simulink model "projeto_bateria_carro_eletrico"  (R2025b)
settings: Solver=VariableStepAuto  StartTime=0.0  StopTime=3600  MaxStep=0.1  RelTol=1e-3
model workspace (MAT data in the model file):
  Fr = 225
  Fr1 = 225
  Fr2 = 450
  Fr3 = 700
  Ft = 1
  V = 100
  t = 4
  v = 38.8888888889
undefined symbols (not defined in the file): Chart, Freio_regenerativo
settings Model: Creator=lucas russo  LastModifiedBy=lucas russo

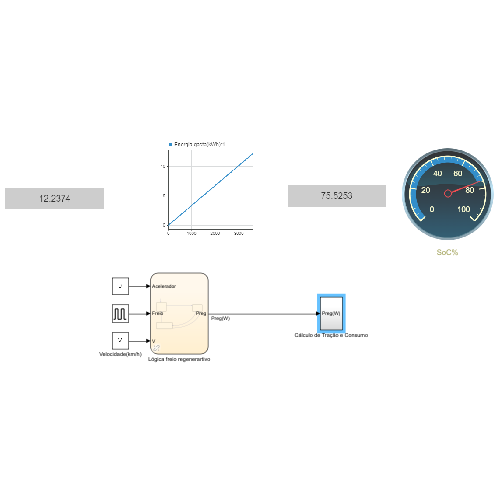
[thumbnail: Simulink's stored preview of the top-level diagram]
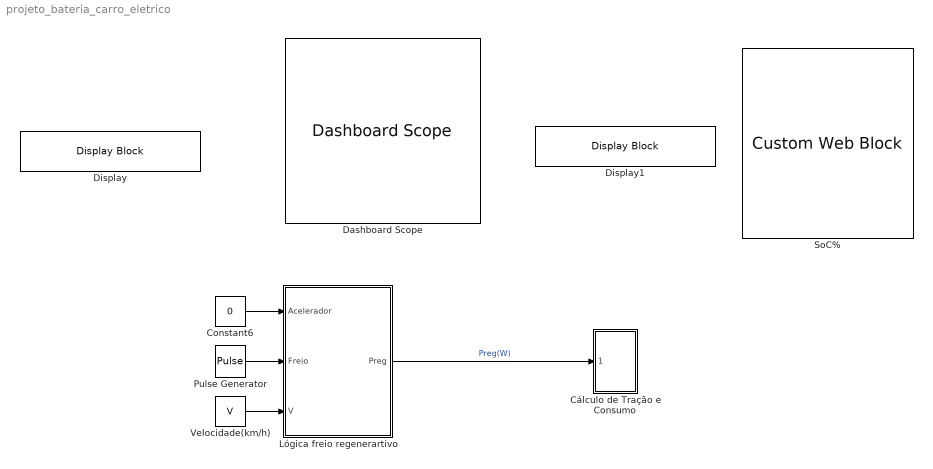
== system projeto_bateria_carro_eletrico ==
  Constant6 : Constant  Value=0
  Cálculo de Tração e Consumo : Subsystem
  Dashboard Scope : DashboardScope  Ymin=0  Ymax=50  FontColor=[0.0, 0.0, 0.0]
  Display : DisplayBlock  LabelPosition=Hide  Transparency=1  GridColor=[0.502, 0.502, 0.502]
  Display1 : DisplayBlock  LabelPosition=Hide  Transparency=1  GridColor=[0.502, 0.502, 0.502]
  Lógica freio regenerartivo : Stateflow chart  AncestorBlock=Freio_regenerativo/Chart
  Pulse Generator : DiscretePulseGenerator  PulseType=Time based  Period=360
  SoC% : CustomWebBlock  LabelPosition=Hide  ShowInitialText=on  Configuration="{\"components\":[{\"name\":\"CircularScaleComponent\",\"settings\":{\"bounds\":{\"max\":100,\"min\":0,\"tickInterval\":\"auto\"},\"direction\":\"cw\",\"flipLimits\":0,\"innerRadius\":0.75,\"internalTickHeightScaleFactor\":1,\"labelColor\":[255,255,200],\"labelFont\":{\"font\":\"Arial\",\"fontSize\":12},\"labelRadius\":0.528,\"labelTransparency\":1,\"minorTickHeightScaleFactor\":0.2,\"needleImage\":{\"size\":[200,50],\"src\":\"data:image\\/svg+xml;base64,PD94bWwgdmVyc2lvbj0iMS4wIiBlbmNvZGluZz0idXRmLTgiPz4KPCEtLSBHZW5lcmF0b3I6IEFkb2JlIElsbHVzdHJhdG9yIDI0LjEuMiwgU1ZHIEV4cG9ydCBQbHVnLUluIC4gU1ZHIFZlcnNpb246IDYuMDAgQnVpbGQgMCkgIC0tPgo8c3ZnIHZlcnNpb249IjEuMSIgaWQ9IkxheWVyXzEiIHhtbG5zPSJodHRwOi8vd3d3LnczLm9yZy8yMDAwL3N2ZyIgeG1sbnM6eGxpbms9Imh0dHA6Ly93d3cudzMub3JnLzE5OTkveGxpbmsiIHg9IjBweCIgeT0iMHB4IgoJIHZpZXdCb3g9IjAgMCAyMDAgNTAiIHN0eWxlPSJlbmFibGUtYmFja2dyb3VuZDpuZXcgMCAwIDIwMCA1MDsiIHhtbDpzcGFjZT0icHJlc2VydmUiPgo8c3R5bGUgdHlwZT0idGV4dC9jc3MiPgoJLnN0MHtmaWxsOiNFQzIxMjc7fQo8L3N0eWxlPgo8cGF0aCBjbGFzcz0ic3QwIiBkPSJNMTYyLjgsMTMuN0MxNjksNC40LDE4MS43LDEuOSwxOTEsOC4xczExLjgsMTguOSw1LjYsMjguMnMtMTguOSwxMS44LTI4LjIsNS42bDAsMAoJQzE1OS4xLDM1LjYsMTU2LjYsMjMsMTYyLjgsMTMuN0wxNjIuOCwxMy43eiBNMTY1LjgsMTUuOGMtNS4xLDcuNi0zLjEsMTcuOSw0LjYsMjNjNy42LDUuMSwxNy45LDMuMSwyMy00LjYKCWM1LjEtNy42LDMuMS0xNy45LTQuNi0yM2wwLDBDMTgxLjIsNi4yLDE3MC45LDguMiwxNjUuOCwxNS44eiIvPgo8cGF0aCBjbGFzcz0ic3QwIiBkPSJNMC40LDI1Ljl2LTMuM2wxNTktMi41Yy0wLjcsMi42LTAuNyw1LjIsMCw3LjhMMC40LDI1Ljl6Ii8+CjxjaXJjbGUgY2xhc3M9InN0MCIgY3g9IjE3OS42IiBjeT0iMjQiIHI9IjAuNyIvPgo8L3N2Zz4K\"},\"needleOffset\":[0.18464878250906522,0],\"needleOrientation\":-45,\"needleRotation\":180,\"needleSize\":{\"height\":0.11741692305346914,\"width\":0.46108337545091255},\"outerRadius\":0.9,\"position\":[0.05,0.05,0.9,0.9],\"referencePoint\":\"auto\",\"scaleAngle\":270,\"scaleAngleOffset\":135,\"scaleColors\":[],\"scaleColorsSize\":0.2,\"scaleDirection\":\"CW\",\"scalePosition\":[0,0,1,1],\"showLabels\":1,\"showMinorTicks\":1,\"showSpanLine\":1,\"showTicks\":1,\"tickColor\":[252,252,197],\"tickTransparency\":1,\"valueBarColor\":[0,114,189],\"valueBarPosition\":[0,0,1,1],\"valueBarSize\":0.2,\"valueBarTransparency\":1}},{\"name\":\"BackgroundImageComponent\",\"settings\":{\"image\":{\"size\":[500,500],\"src\":\"data:image\\/svg+xml;base64,PD94bWwgdmVyc2lvbj0iMS4wIiBlbmNvZGluZz0iVVRGLTgiIHN0YW5kYWxvbmU9Im5vIj8+CjxzdmcKICAgeG1sbnM6ZGM9Imh0dHA6Ly9wdXJsLm9yZy9kYy9lbGVtZW50cy8xLjEvIgogICB4bWxuczpjYz0iaHR0cDovL2NyZWF0aXZlY29tbW9ucy5vcmcvbnMjIgogICB4bWxuczpyZGY9Imh0dHA6Ly93d3cudzMub3JnLzE5OTkvMDIvMjItcmRmLXN5bnRheC1ucyMiCiAgIHhtbG5zOnN2Zz0iaHR0cDovL3d3dy53My5vcmcvMjAwMC9zdmciCiAgIHhtbG5zPSJodHRwOi8vd3d3LnczLm9yZy8yMDAwL3N2ZyIKICAgeG1sbnM6 ...(+9964 chars)\"},\"position\":[0,0,1,1],\"scaleMode\":\"0\"}},{\"name\":\"ForegroundImageComponent\",\"settings\":{\"image\":{\"size\":[0,0],\"src\":\"default\",\"srcOrientation\":[]},\"isForeground\":1,\"position\":[0,0,1,1],\"scaleMode\":\"0\"}}],\"derived\":{\"blockParameters\":{\"ForegroundColor\":[0.9882352941176471,0.9882352941176471,0.7725490196078432],\"Limits\":{\"Max\":100,\"Min\":0,\"Ticks\":\"auto\"},\"ScaleColors\":[],\"ScaleDirection\":\"Clockwise\",\"ScaleMax\":100,\"ScaleMin\":0,\"TickInterval\":\"auto\",\"fixedAspectRatio\":\"on\"}},\"settings\":{\"BindingType\":\"signal\",\"aspectRatio\":1.032258064516129,\"backgroundColor\":[0,0,0,\"1\"],\"backgroundOffset\":1,\"backgroundOpacity\":1,\"direction\":\"cw\",\"fixedAspectRatio\":\"on\",\"flipLimits\":0,\"orientation\":\"horizontal\",\"showBackgroundColor\":false,\"value\":0,\"version\":\"R2023a\"},\"type\":\"CircularGauge\"}"
  Velocidade(km/h) : Constant  Value=V
  wires:
  Pulse Generator/1 -> Lógica freio regenerartivo/2(Freio)
  Velocidade(km/h)/1 -> Lógica freio regenerartivo/3(V)
  Constant6/1 -> Lógica freio regenerartivo/1(Acelerador)
  Lógica freio regenerartivo/1(Preg) -> Cálculo de Tração e Consumo/1(Preg(W))  "Preg(W)"

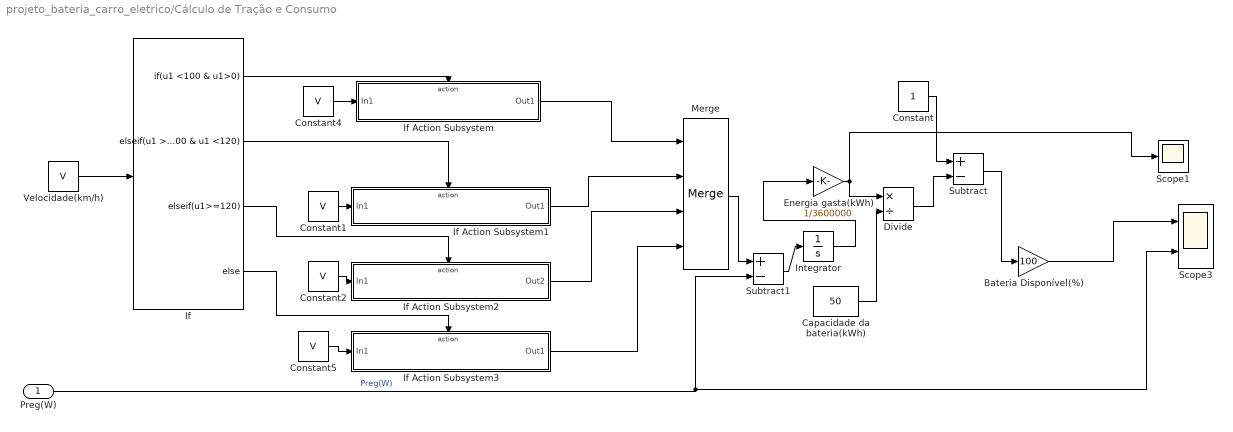
== system projeto_bateria_carro_eletrico/Cálculo de Tração e Consumo ==
  Preg(W) : Inport
  Bateria Disponível(%) : Gain  Gain=100
  Capacidade da bateria(kWh) : Constant  Value=50
  Constant : Constant
  Constant{1..2,4..5} (4 alike) : Constant  Value=V
  Divide : Product  Inputs=*/
  Energia gasta(kWh) : Gain  Gain=1/3600000
  If : If  IfExpression=u1 <100 & u1>0  ElseIfExpressions=u1 >=100 & u1 <120,u1>=120
  If Action Subsystem : Subsystem  TreatAsAtomicUnit=on
  If Action Subsystem1 : Subsystem  TreatAsAtomicUnit=on
  If Action Subsystem2 : Subsystem  TreatAsAtomicUnit=on
  If Action Subsystem3 : Subsystem  TreatAsAtomicUnit=on
  Integrator : Integrator  UpperSaturationLimit=100  LowerSaturationLimit=0
  Merge : Merge  Inputs=4
  Scope1 : Scope
      settings: ActiveDisplayYMinimum=10.624641425804962  ActiveDisplayYMaximum=11.300685063058687
  Scope3 : Scope  NumInputPorts=2
      settings: ActiveDisplayYMinimum=87.23903917985831  ActiveDisplayYMaximum=87.881272359204075  DataLoggingVariableName=ScopeData3
  Subtract : Sum  Inputs=+-
  Subtract1 : Sum  Inputs=+-
  Velocidade(km/h) : Constant  Value=V
  wires:
  If/2 -> If Action Subsystem1/Action
  Energia gasta(kWh)/1 -> Scope1/1, Divide/1
  Constant/1 -> Subtract/1
  Constant1/1 -> If Action Subsystem1/1(In1)
  Divide/1 -> Subtract/2
  If/4 -> If Action Subsystem3/Action
  Capacidade da bateria(kWh)/1 -> Divide/2
  Velocidade(km/h)/1 -> If/1
  If Action Subsystem1/1(Out1) -> Merge/2
  If Action Subsystem3/1(Out1) -> Merge/4
  Constant4/1 -> If Action Subsystem/1(In1)
  If/3 -> If Action Subsystem2/Action
  If Action Subsystem2/1(Out2) -> Merge/3
  If/1 -> If Action Subsystem/Action
  Constant5/1 -> If Action Subsystem3/1(In1)
  If Action Subsystem/1(Out1) -> Merge/1
  Constant2/1 -> If Action Subsystem2/1(In1)
  Subtract/1 -> Bateria Disponível(%)/1
  Merge/1 -> Subtract1/1
  Preg(W)/1 -> Scope3/2, Subtract1/2  "Preg(W)"
  Subtract1/1 -> Integrator/1
  Integrator/1 -> Energia gasta(kWh)/1
  Bateria Disponível(%)/1 -> Scope3/1

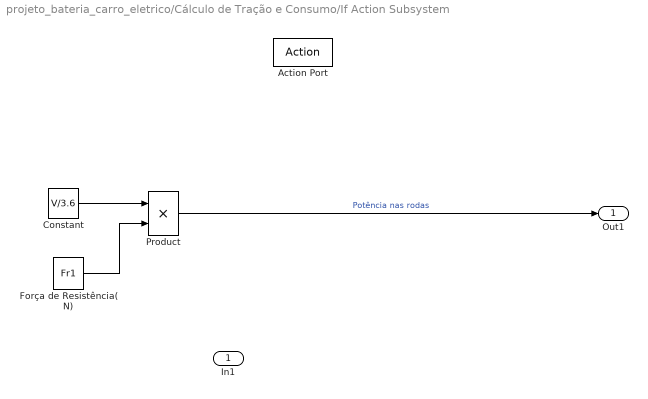
== system projeto_bateria_carro_eletrico/Cálculo de Tração e Consumo/If Action Subsystem ==
  In1 : Inport
  Action Port : ActionPort  ActionPortLabel=if(u1 <100 & u1>0)
  Constant : Constant  Value=V/3.6
  Força de Resistência(N) : Constant  Value=Fr1
  Product : Product
  Out1 : Outport
  wires:
  Força de Resistência(N)/1 -> Product/2
  Constant/1 -> Product/1
  Product/1 -> Out1/1  "Potência nas rodas"

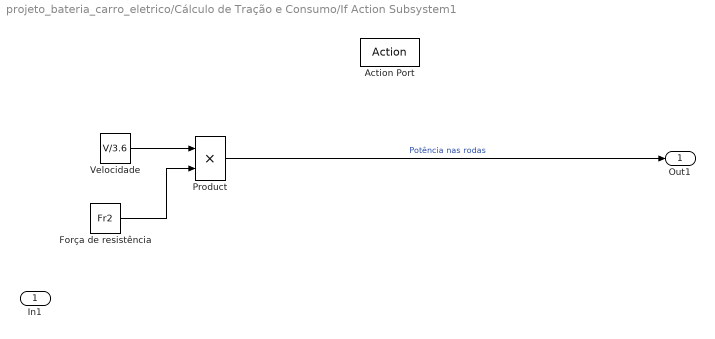
== system projeto_bateria_carro_eletrico/Cálculo de Tração e Consumo/If Action Subsystem1 ==
  In1 : Inport
  Action Port : ActionPort  ActionPortLabel=elseif(u1 >=100 & u1 <120)
  Força de resistência : Constant  Value=Fr2
  Product : Product
  Velocidade : Constant  Value=V/3.6
  Out1 : Outport
  wires:
  Força de resistência/1 -> Product/2
  Velocidade/1 -> Product/1
  Product/1 -> Out1/1  "Potência nas rodas"

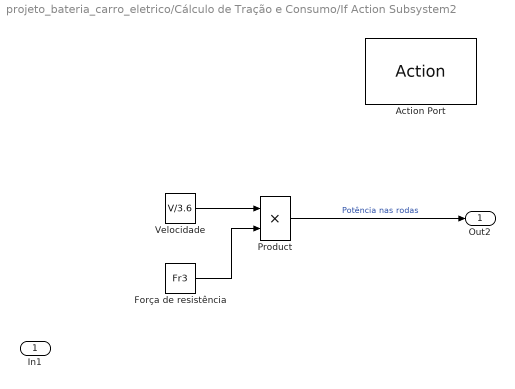
== system projeto_bateria_carro_eletrico/Cálculo de Tração e Consumo/If Action Subsystem2 ==
  In1 : Inport
  Action Port : ActionPort  ActionPortLabel=elseif(u1>=120)
  Força de resistência : Constant  Value=Fr3
  Product : Product
  Velocidade : Constant  Value=V/3.6
  Out2 : Outport
  wires:
  Força de resistência/1 -> Product/2
  Velocidade/1 -> Product/1
  Product/1 -> Out2/1  "Potência nas rodas"

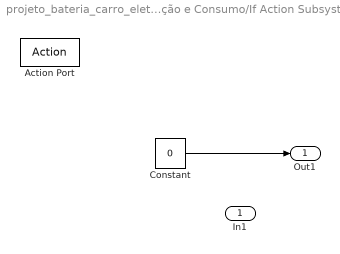
== system projeto_bateria_carro_eletrico/Cálculo de Tração e Consumo/If Action Subsystem3 ==
  In1 : Inport
  Action Port : ActionPort  ActionPortLabel=else
  Constant : Constant  Value=0
  Out1 : Outport
  wires:
  Constant/1 -> Out1/1

== stateflow chart projeto_bateria_carro_eletrico/Lógica freio regenerartivo ==
  state Aceleracao
    during:
    Preg=0;
  state Inercia
    during:
    Preg=0;
  state Frenagem
    during:
    Preg= (V/3.6) *0.7 * 1500;
  (default) -> Aceleracao
  Aceleracao -> Inercia : [Acelerador<=0.01 & Freio==0]
  Frenagem -> Aceleracao [order 1] : [Acelerador>0]
  Inercia -> Frenagem : [Freio>0 & V>5]
  Frenagem -> Inercia [order 2] : [Freio==0 | V<=5]
  data: Acelerador input; Freio input; Preg output; V input
